simulink library "mssSimulink"  (R2024a)
settings: Solver=ode45  StartTime=0.0  StopTime=10.0  RelTol=1e-3
undefined symbols (not defined in the file): ABC, CN_data, CX_data, CY_data, D, G, Hoerner, K_supply, kt2ms, MA, magnitude, MRB, pathlength, RAO_Amp, RAO_Dir, RAO_Freq, RAO_Phase, RAO_Vel, RAO_yaw_back, RAO_yaw_quant, RAO_yaw_quantization_flag, rho_a, slcm, T_supply, table, vessel, vesselABC
libraries: $bdroot x99, simulink x13
(part 3 of 9)

== system mssSimulink/Hydrodynamics/Motion RAO (U=0) ==
  eta LF : Inport
  Waves : Inport  Port=2
  6DOF rotation matrix in yaw : Subsystem
  Bus Selector : BusSelector  OutputSignals=Psi,Wavenum,Omega,Phase,Zeta_a
  Clock : Clock
  Output smoothing : Subsystem
  "Position phase " : $bdroot/Modelling/Environmental Loads/Utilities/Position phase
  Product1 : Product  Inputs=**  SaturateOnIntegerOverflow=on  OutDataTypeStr=Inherit: Same as first input
  Sum : Sum  Inputs=-++  SaturateOnIntegerOverflow=on
  Wave component loop : Subsystem  TreatAsAtomicUnit=on
  Width : Width  DataType=int32
  "Yaw quantizer " : $bdroot/Modelling/Environmental Loads/Utilities/Yaw quantizer  quant_flag=RAO_yaw_quantization_flag  quant=RAO_yaw_quant  back=RAO_yaw_back
  "[-inf inf] to [-pi pi] " : $bdroot/Utilities/Math Operations/[-inf inf] to [-pi pi]
  yaw angle : Selector  InputPortWidth=6  IndexOptions=Index vector (dialog)  Indices=6  OutputSizes=1
  eta WF : Outport
  nu WF : Outport  Port=2
  nu_dot WF : Outport  Port=3
  wires:
  Output smoothing/1("eta_h WF ") -> 6DOF rotation matrix in yaw/2(V)
  Wave component loop/4(nu_dot rate) -> Output smoothing/4(nu_dot rate)
  Wave component loop/1(eta_h WF) -> Output smoothing/1(eta_h WF)
  Output smoothing/3(nu_dot WF) -> nu_dot WF/1
  Output smoothing/2(nu WF) -> nu WF/1
  eta LF/1 -> yaw angle/1, "Position phase "/3
  Bus Selector/2 -> "Position phase "/2  "<Wavenum>"
  Bus Selector/4 -> Sum/3  "<Phase>"
  Waves/1 -> Bus Selector/1
  Product1/1 -> Sum/2
  Bus Selector/1 -> "Position phase "/1, "Yaw quantizer "/2  "<Psi>"
  Clock/1 -> Product1/2
  yaw angle/1 -> 6DOF rotation matrix in yaw/1(psi), "Yaw quantizer "/1
  Bus Selector/3 -> Width/1, Wave component loop/3(Omega), Product1/1  "<Omega>"
  6DOF rotation matrix in yaw/1(R(psi)*V) -> eta WF/1
  Sum/1 -> Wave component loop/4(Phase_tot)  "Phase_tot"
  Bus Selector/5 -> Wave component loop/5(Zeta_a)  "<Zeta_a>"
  Width/1 -> Wave component loop/1(number of iterations)
  Wave component loop/2(nu WF) -> Output smoothing/2("nu WF ")
  Wave component loop/3(nu_dot WF) -> Output smoothing/3("nu_dot WF ")
  "Yaw quantizer "/1 -> "[-inf inf] to [-pi pi] "/1
  "[-inf inf] to [-pi pi] "/1 -> Wave component loop/2(Psi_r)
  "Position phase "/1 -> Sum/1

== system mssSimulink/Hydrodynamics/WD for heading1 ==
  psi : Inport
  psi_wave : Inport  Port=2
  Omega : Inport  Port=3
  Zeta_a : Inport  Port=4
  U : Inport  Port=5
  Sum1 : Sum  Inputs=-+|
  Wave component loop : Subsystem  TreatAsAtomicUnit=on
  Width : Width  DataType=int32
  tau_WD : Outport
  wires:
  Width/1 -> Wave component loop/1(number of iterations)
  psi_wave/1 -> Sum1/2
  Omega/1 -> Wave component loop/3(Omega), Width/1
  Zeta_a/1 -> Wave component loop/4(Zeta_a)
  Sum1/1 -> Wave component loop/2(Psi_r)
  Wave component loop/1(tau_WD) -> tau_WD/1
  U/1 -> Wave component loop/5(U)
  psi/1 -> Sum1/1  "psi"

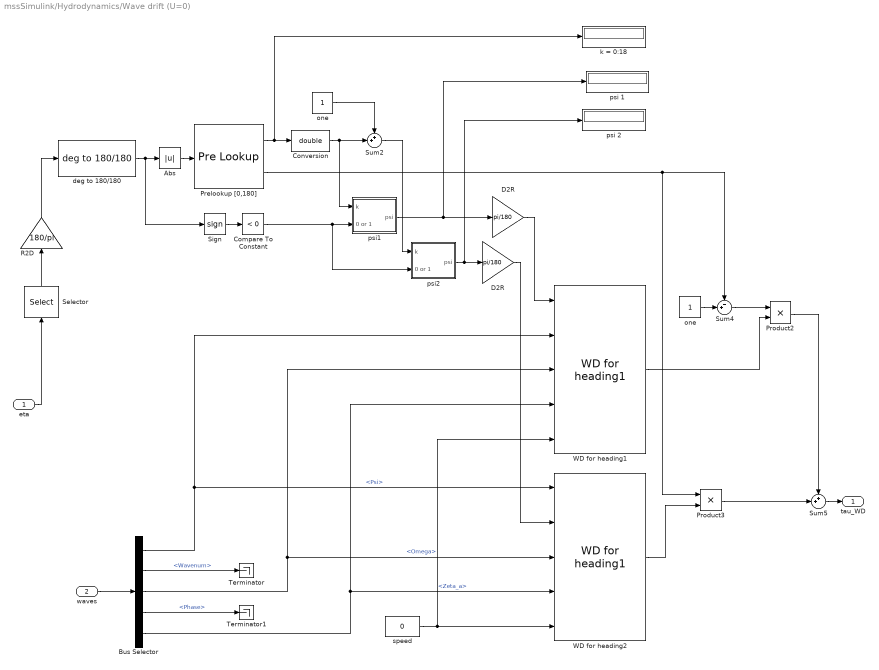
== system mssSimulink/Hydrodynamics/Wave drift (U=0) ==
  eta : Inport
  waves : Inport  Port=2
  Abs : Abs
  Bus Selector : BusSelector  OutputSignals=Psi,Wavenum,Omega,Phase,Zeta_a
  Compare To Constant : simulink/Logic and Bit Operations/Compare To Constant  relop=<  const=0  OutDataTypeStr=uint8  ZeroCross=off
  Conversion : DataTypeConversion  OutDataTypeStr=double  SaturateOnIntegerOverflow=off  RndMeth=Floor
  D2R : Gain  Gain=pi/180
  "D2R " : Gain  Gain=pi/180
  Prelookup [0,180] : PreLookup  BreakpointsData=[0:10:180]  IndexSearchMethod=Evenly spaced points  BeginIndexSearchUsingPreviousIndexResult=on
  Product2 : Product  RndMeth=Zero
  Product3 : Product  RndMeth=Zero
  R2D : Gain  Gain=180/pi
  Selector : Selector  InputPortWidth=6  IndexOptions=Index vector (dialog)  Indices=[6]  OutputSizes=1
  Sign : Signum
  Sum2 : Sum  Inputs=++|
  Sum4 : Sum  Inputs=-+|
  Sum5 : Sum  Inputs=++|
  Terminator : Terminator
  Terminator1 : Terminator
  "WD for heading1 " : $bdroot/Hydrodynamics/WD for heading1  ForceRAO_Freq=vessel.forceRAO.w  WD_Freq=vessel.driftfrc.w  RAO_Vel=vessel.velocities  ForceRAO_Amp=vessel.forceRAO.amp  ForceRAO_Phase=vessel.forceRAO.phase  WD_Amp=vessel.driftfrc.amp  RAO_add_omega_0=on  RAO_add_omega_inf=on
  "WD for heading2 " : $bdroot/Hydrodynamics/WD for heading1  ForceRAO_Freq=vessel.forceRAO.w  WD_Freq=vessel.driftfrc.w  RAO_Vel=vessel.velocities  ForceRAO_Amp=vessel.forceRAO.amp  ForceRAO_Phase=vessel.forceRAO.phase  WD_Amp=vessel.driftfrc.amp  RAO_add_omega_0=on  RAO_add_omega_inf=on
  "deg to 180/180 " : $bdroot/Utilities/Math Operations/deg to 180//180
  k = 0:18 : Display
  one : Constant
  "one " : Constant
  psi 1 : Display
  psi 2 : Display
  psi1 : Subsystem
  psi2 : Subsystem
  speed : Constant  Value=0
  tau_WD : Outport
  wires:
  "WD for heading2 "/1 -> Product3/2
  eta/1 -> Selector/1
  "one "/1 -> Sum4/2
  Sum4/1 -> Product2/1
  "WD for heading1 "/1 -> Product2/2
  Product3/1 -> Sum5/2
  Product2/1 -> Sum5/1
  Prelookup [0,180]/1 -> Conversion/1, k = 0:18/1
  one/1 -> Sum2/1
  Sum2/1 -> psi2/1(k)
  "deg to 180/180 "/1 -> Abs/1, Sign/1
  Abs/1 -> Prelookup [0,180]/1
  Sign/1 -> Compare To Constant/1
  Compare To Constant/1 -> psi1/2(0 or 1), psi2/2(0 or 1)
  psi1/1(psi) -> D2R/1, psi 1/1
  Prelookup [0,180]/2 -> Product3/1, Sum4/1
  Conversion/1 -> Sum2/2, psi1/1(k)
  psi2/1(psi) -> "D2R "/1, psi 2/1
  waves/1 -> Bus Selector/1
  Sum5/1 -> tau_WD/1
  Selector/1 -> R2D/1
  R2D/1 -> "deg to 180/180 "/1
  speed/1 -> "WD for heading2 "/5, "WD for heading1 "/5
  Bus Selector/3 -> "WD for heading2 "/3, "WD for heading1 "/3  "<Omega>"
  Bus Selector/5 -> "WD for heading2 "/4, "WD for heading1 "/4  "<Zeta_a>"
  Bus Selector/2 -> Terminator/1  "<Wavenum>"
  Bus Selector/1 -> "WD for heading1 "/2, "WD for heading2 "/1  "<Psi>"
  Bus Selector/4 -> Terminator1/1  "<Phase>"
  D2R/1 -> "WD for heading1 "/1
  "D2R "/1 -> "WD for heading2 "/2

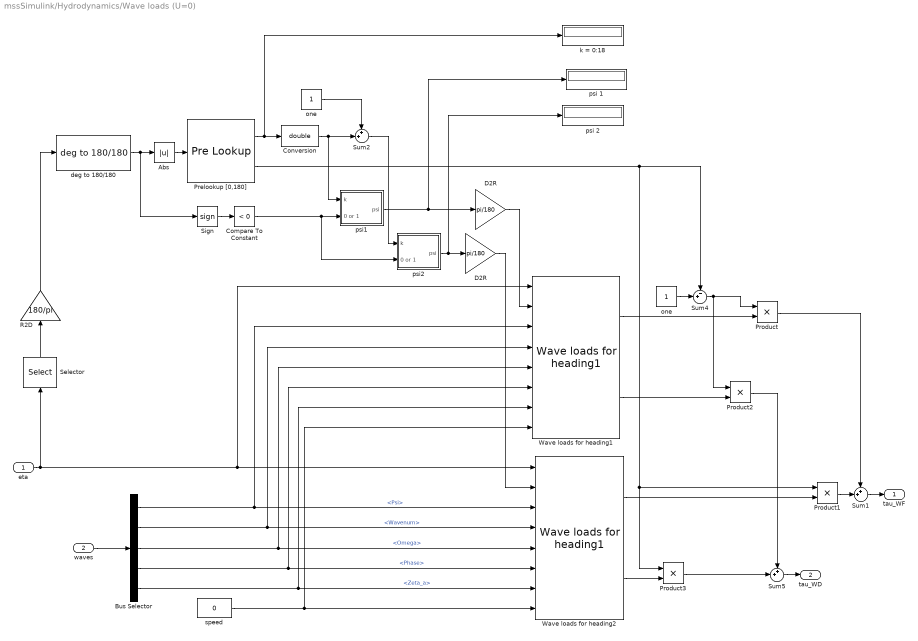
== system mssSimulink/Hydrodynamics/Wave loads (U=0) ==
  eta : Inport
  waves : Inport  Port=2
  Abs : Abs
  Bus Selector : BusSelector  OutputSignals=Psi,Wavenum,Omega,Phase,Zeta_a
  Compare To Constant : simulink/Logic and Bit Operations/Compare To Constant  relop=<  const=0  OutDataTypeStr=uint8  ZeroCross=off
  Conversion : DataTypeConversion  OutDataTypeStr=double  SaturateOnIntegerOverflow=off  RndMeth=Floor
  D2R : Gain  Gain=pi/180
  "D2R " : Gain  Gain=pi/180
  Prelookup [0,180] : PreLookup  BreakpointsData=[0:10:180]  IndexSearchMethod=Evenly spaced points  BeginIndexSearchUsingPreviousIndexResult=on
  Product{,1..3} (4 alike) : Product  RndMeth=Zero
  R2D : Gain  Gain=180/pi
  Selector : Selector  InputPortWidth=6  IndexOptions=Index vector (dialog)  Indices=[6]  OutputSizes=1
  Sign : Signum
  Sum1 : Sum  Inputs=++|
  Sum2 : Sum  Inputs=++|
  Sum4 : Sum  Inputs=-+|
  Sum5 : Sum  Inputs=++|
  "Wave loads for heading1 " : $bdroot/Hydrodynamics/Wave loads for heading1  ForceRAO_Freq=vessel.forceRAO.w  WD_Freq=vessel.driftfrc.w  RAO_Vel=vessel.velocities  ForceRAO_Amp=vessel.forceRAO.amp  ForceRAO_Phase=vessel.forceRAO.phase  WD_Amp=vessel.driftfrc.amp  RAO_add_omega_0=on  RAO_add_omega_inf=on
  Wave loads for heading2 : $bdroot/Hydrodynamics/Wave loads for heading1  ForceRAO_Freq=vessel.forceRAO.w  WD_Freq=vessel.driftfrc.w  RAO_Vel=vessel.velocities  ForceRAO_Amp=vessel.forceRAO.amp  ForceRAO_Phase=vessel.forceRAO.phase  WD_Amp=vessel.driftfrc.amp  RAO_add_omega_0=on  RAO_add_omega_inf=on
  "deg to 180/180 " : $bdroot/Utilities/Math Operations/deg to 180//180
  k = 0:18 : Display
  one : Constant
  "one " : Constant
  psi 1 : Display
  psi 2 : Display
  psi1 : Subsystem
  psi2 : Subsystem
  speed : Constant  Value=0
  tau_WF : Outport
  tau_WD : Outport  Port=2
  wires:
  R2D/1 -> "deg to 180/180 "/1
  Selector/1 -> R2D/1
  Sum5/1 -> tau_WD/1
  waves/1 -> Bus Selector/1
  Sum1/1 -> tau_WF/1
  "D2R "/1 -> Wave loads for heading2/2
  D2R/1 -> "Wave loads for heading1 "/2
  psi2/1(psi) -> psi 2/1, "D2R "/1
  Conversion/1 -> psi1/1(k), Sum2/2
  Prelookup [0,180]/2 -> Sum4/1, Product1/1, Product3/1
  psi1/1(psi) -> psi 1/1, D2R/1
  Compare To Constant/1 -> psi2/2(0 or 1), psi1/2(0 or 1)
  Sign/1 -> Compare To Constant/1
  Abs/1 -> Prelookup [0,180]/1
  "deg to 180/180 "/1 -> Sign/1, Abs/1
  Sum2/1 -> psi2/1(k)
  one/1 -> Sum2/1
  Prelookup [0,180]/1 -> k = 0:18/1, Conversion/1
  Product2/1 -> Sum5/1
  Product3/1 -> Sum5/2
  "Wave loads for heading1 "/2 -> Product2/2
  Sum4/1 -> Product2/1, Product/1
  "one "/1 -> Sum4/2
  Product1/1 -> Sum1/2
  Product/1 -> Sum1/1
  "Wave loads for heading1 "/1 -> Product/2
  Bus Selector/5 -> Wave loads for heading2/7, "Wave loads for heading1 "/7  "<Zeta_a>"
  Bus Selector/4 -> Wave loads for heading2/6, "Wave loads for heading1 "/6  "<Phase>"
  Bus Selector/3 -> Wave loads for heading2/5, "Wave loads for heading1 "/5  "<Omega>"
  Bus Selector/2 -> Wave loads for heading2/4, "Wave loads for heading1 "/4  "<Wavenum>"
  Bus Selector/1 -> Wave loads for heading2/3, "Wave loads for heading1 "/3  "<Psi>"
  eta/1 -> Selector/1, Wave loads for heading2/1, "Wave loads for heading1 "/1
  Wave loads for heading2/2 -> Product3/2
  Wave loads for heading2/1 -> Product1/2
  speed/1 -> Wave loads for heading2/8, "Wave loads for heading1 "/8

== system mssSimulink/Hydrodynamics/Wave loads (U>0) ==
  eta : Inport
  waves : Inport  Port=2
  U : Inport  Port=3
  Abs : Abs
  Conversion : DataTypeConversion  OutDataTypeStr=double  SaturateOnIntegerOverflow=off  RndMeth=Floor
  Prelookup : PreLookup  BreakpointsData=vessel.velocities  IndexSearchMethod=Linear search  BeginIndexSearchUsingPreviousIndexResult=on
  Product{,1..3} (4 alike) : Product  RndMeth=Zero
  Sum1 : Sum  Inputs=++|
  Sum2 : Sum  Inputs=++|
  Sum4 : Sum  Inputs=-+|
  Sum5 : Sum  Inputs=++|
  Wave loads U = U1 : Subsystem
  Wave loads U = U2 : Subsystem
  one : Constant
  "one " : Constant
  tau_WF : Outport
  tau_WD : Outport  Port=2
  wires:
  waves/1 -> Wave loads U = U1/2(waves), Wave loads U = U2/2(waves)
  eta/1 -> Wave loads U = U1/1(eta), Wave loads U = U2/1(eta)
  Conversion/1 -> Sum2/2, Wave loads U = U1/3(U_idx)
  Abs/1 -> Prelookup/1
  one/1 -> Sum2/1
  Prelookup/1 -> Conversion/1
  Sum2/1 -> Wave loads U = U2/3(U_idx)
  Sum5/1 -> tau_WD/1
  Sum1/1 -> tau_WF/1
  Prelookup/2 -> Product1/1, Product3/1, Sum4/1
  Product2/1 -> Sum5/1
  Product3/1 -> Sum5/2
  Sum4/1 -> Product2/1, Product/1
  "one "/1 -> Sum4/2
  Product1/1 -> Sum1/2
  Product/1 -> Sum1/1
  Wave loads U = U1/1(tau_WF) -> Product/2
  Wave loads U = U2/2(tau_WD) -> Product3/2
  Wave loads U = U2/1(tau_WF) -> Product1/2
  Wave loads U = U1/2(tau_WD) -> Product2/2
  U/1 -> Abs/1

== system mssSimulink/Hydrodynamics/Wave loads for heading1 ==
  eta : Inport
  psi : Inport  Port=2
  psi_wave : Inport  Port=3
  wavenum : Inport  Port=4
  Omega : Inport  Port=5
  Phase : Inport  Port=6
  Zeta_a : Inport  Port=7
  U : Inport  Port=8
  Clock : Clock
  "Position phase " : $bdroot/Modelling/Environmental Loads/Utilities/Position phase
  Product1 : Product  Inputs=**  SaturateOnIntegerOverflow=on  OutDataTypeStr=Inherit: Same as first input
  Sum : Sum  Inputs=-++  SaturateOnIntegerOverflow=on
  Sum1 : Sum  Inputs=-+|
  Wave component loop : Subsystem  TreatAsAtomicUnit=on
  Width : Width  DataType=int32
  tau_WF : Outport
  tau_WD : Outport  Port=2
  wires:
  psi/1 -> Sum1/1  "psi"
  U/1 -> Wave component loop/6(U)
  Wave component loop/2(tau_WD) -> tau_WD/1
  Sum1/1 -> Wave component loop/2(Psi_r)
  Zeta_a/1 -> Wave component loop/5(Zeta_a)
  Phase/1 -> Sum/3
  Omega/1 -> Width/1, Wave component loop/3(Omega), Product1/1
  wavenum/1 -> "Position phase "/2
  psi_wave/1 -> Sum1/2, "Position phase "/1
  eta/1 -> "Position phase "/3
  Wave component loop/1(tau_WF) -> tau_WF/1
  Product1/1 -> Sum/2
  Clock/1 -> Product1/2
  Sum/1 -> Wave component loop/4(Phase_tot)  "Phase_tot"
  Width/1 -> Wave component loop/1(number of iterations)
  "Position phase "/1 -> Sum/1

== system mssSimulink/Hydrodynamics/zero-speed viiscous roll damping ==
  p : Inport
  A44 : Constant  Value=vesselABC.A44(:,:,1)
  B44 : Constant  Value=vesselABC.B44(:,:,1)
  B44_inf : Constant  Value=vesselABC.B44_inf(1)
  C44 : Constant  Value=vesselABC.C44(:,:,1)
  D44 : Constant  Value=vesselABC.D44(:,:,1)
  Integrator : Integrator
  Math Function : Math  Operator=transpose  SignedPower=on
  Product{,1..2,4} (4 alike) : Product  Multiplication=Matrix(*)  RndMeth=Zero
  Product3 : Product  RndMeth=Zero
  Sum : Sum  Inputs=++|
  Sum1 : Sum  Inputs=|++
  Sum2 : Sum  Inputs=++|
  K_visc : Outport
  wires:
  Math Function/1 -> Product2/1
  B44/1 -> Product1/1
  Sum1/1 -> Sum2/2
  Product2/1 -> Sum1/1
  Product3/1 -> Sum1/2
  D44/1 -> Product3/1
  C44/1 -> Math Function/1
  Sum/1 -> Integrator/1
  Product/1 -> Sum/2
  Product1/1 -> Sum/1
  A44/1 -> Product/1
  Integrator/1 -> Product2/2, Product/2
  p/1 -> Product3/2, Product1/2, Product4/2
  Sum2/1 -> K_visc/1
  B44_inf/1 -> Product4/1
  Product4/1 -> Sum2/1

== system mssSimulink/Marine craft models/4-DOF naval vessel ==
  tau (X,Y,K,N) : Inport
  Initial conditions (u,v,p,r,phi,psi) : Constant  Value=x0
  Integrator : Integrator  InitialConditionSource=external  InitialCondition=[1 1]  UpperSaturationLimit=10  LowerSaturationLimit=-10
  Mux1 : Mux  Inputs=2
  Selector : Selector  InputPortWidth=6  IndexOptions=Index vector (dialog)  Indices=[1 2 3 4]  OutputSizes=1
  Selector1 : Selector  InputPortWidth=6  IndexOptions=Index vector (dialog)  Indices=[5 6]  OutputSizes=1
  navalvessel.m : MATLABFcn  MATLABFcn=feval('navalvessel',u(1:6),u(7:10))  OutputDimensions=6  Output1D=off
  eta (phi,psi) : Outport  VectorParamsAs1DForOutWhenUnconnected=off
  nu (u,v,p,r) : Outport  Port=2  VectorParamsAs1DForOutWhenUnconnected=off
  wires:
  Selector/1 -> nu (u,v,p,r)/1
  Selector1/1 -> eta (phi,psi)/1
  Integrator/1 -> Selector1/1, Selector/1, Mux1/1
  Initial conditions (u,v,p,r,phi,psi)/1 -> Integrator/2
  tau (X,Y,K,N)/1 -> Mux1/2
  navalvessel.m/1 -> Integrator/1
  Mux1/1 -> navalvessel.m/1

== system mssSimulink/Marine craft models/6-DOF semisub ==
  tau : Inport
  nu_c : Inport  Port=2
  "6 DOF Eqs. of motion " : $bdroot/Modelling/Kinetics /6 DOF Eqs. of motion  CoriolisOnOff=on  nu0=[0 0 0 0 0 0]  eta0=[0 0 0 0 0 0]
      link override 6 DOF Coriolis forces: SourceBlock=mssSimulink/Modelling/Kinetics /Support/6 DOF Coriolis forces
      link override 6 DOF Coriolis forces1: SourceBlock=mssSimulink/Modelling/Kinetics /Support/6 DOF Coriolis forces
      link override Euler angles to rotation matrix: SourceBlock=mssSimulink/Modelling/Kinematics/Euler angles to rotation matrix
  Constant : Constant  Value=MRB
  "Constant " : Constant  Value=MA
  D : Gain  Gain=D  Multiplication=Matrix(K*u)  SaturateOnIntegerOverflow=on  OutDataTypeStr=Inherit: Same as input  ParamDataTypeStr=Inherit: Same as input
  G : Gain  Gain=G  Multiplication=Matrix(K*u)  SaturateOnIntegerOverflow=on  OutDataTypeStr=Inherit: Same as input  ParamDataTypeStr=Inherit: Same as input
  Sum : Sum  Inputs=+--  InputSameDT=on  SaturateOnIntegerOverflow=on  OutDataTypeStr=Inherit: Same as first input
  Sum1 : Sum  Inputs=-+|  SaturateOnIntegerOverflow=on
  eta : Outport  InitialOutput=0  VectorParamsAs1DForOutWhenUnconnected=off
  nu : Outport  Port=2  InitialOutput=0  VectorParamsAs1DForOutWhenUnconnected=off
  wires:
  "Constant "/1 -> "6 DOF Eqs. of motion "/2
  Sum/1 -> "6 DOF Eqs. of motion "/3
  Sum1/1 -> D/1
  nu_c/1 -> Sum1/1, "6 DOF Eqs. of motion "/4
  Constant/1 -> "6 DOF Eqs. of motion "/1
  "6 DOF Eqs. of motion "/1 -> eta/1, G/1
  "6 DOF Eqs. of motion "/2 -> Sum1/2, nu/1
  G/1 -> Sum/2
  D/1 -> Sum/3
  tau/1 -> Sum/1

== system mssSimulink/Marine craft models/6-DOF supply vessel interface ==
  tau : Inport
  3 to 6 DOF : $bdroot/Modelling/Kinetics /Support/3 to 6 DOF  SystemSampleTime=-1  VariantActivationTime=update diagram  AllowFlexibleInterface=on  Latency=0  AutoFrameSizeCalculation=off
  3 to 6 DOF1 : $bdroot/Modelling/Kinetics /Support/3 to 6 DOF  SystemSampleTime=-1  VariantActivationTime=update diagram  AllowFlexibleInterface=on  Latency=0  AutoFrameSizeCalculation=off
  6 to 3 DOF1 : Selector  InputPortWidth=6  IndexOptions=Index vector (dialog)  Indices=[1 2 6]  OutputSizes=1
  Supply vessel : $bdroot/Marine craft models/Supply vessel  D=[5.0242e4 0 0; 0 2.7229e5 -4.3933e6; 0 -4.3933e6 4.1894e8]  Minv=inv( [5.3122e6 0 0; 0 8.2831e6 0; 0 0 3.7454e9] )
  eta : Outport  VectorParamsAs1DForOutWhenUnconnected=off
  nu : Outport  Port=2  VectorParamsAs1DForOutWhenUnconnected=off
  wires:
  3 to 6 DOF1/1 -> nu/1
  tau/1 -> 6 to 3 DOF1/1
  3 to 6 DOF/1 -> eta/1
  6 to 3 DOF1/1 -> Supply vessel/1
  Supply vessel/2 -> 3 to 6 DOF1/1
  Supply vessel/1 -> 3 to 6 DOF/1

== system mssSimulink/Marine craft models/Container ship: L = 175 m ==
  u : Inport
  xo : Inport  Port=2
  Integrator : Integrator  InitialConditionSource=external  InitialCondition=[1 1]  UpperSaturationLimit=10  LowerSaturationLimit=-10
  Mux1 : Mux  Inputs=2
  m-file : MATLABFcn  MATLABFcn=feval(vessmodel,u(1:dimx_model),u(dimx_model+1:length(u)))  Output1D=off
  x : Outport  VectorParamsAs1DForOutWhenUnconnected=off
  wires:
  xo/1 -> Integrator/2
  u/1 -> Mux1/2
  Mux1/1 -> m-file/1
  Integrator/1 -> x/1, Mux1/1
  m-file/1 -> Integrator/1

== system mssSimulink/Marine craft models/CyberShipII ==
  note: etadot
  note: nu_dot
  note: nu
  tau : Inport
  D : Gain  Gain=D  Multiplication=Matrix(K*u)  SaturateOnIntegerOverflow=on  OutDataTypeStr=Inherit: Same as input  ParamDataTypeStr=Inherit: Same as input
  Integrator1 : Integrator
  Integrator2 : Integrator
  Rotation matrix in yaw 1 : $bdroot/Modelling/Kinematics/Rotation matrix in yaw 
  Sum3 : Sum  Inputs=+-  InputSameDT=on  SaturateOnIntegerOverflow=on  OutDataTypeStr=Inherit: Same as first input
  inv(M) : Gain  Gain=inv(M)  Multiplication=Matrix(K*u)  SaturateOnIntegerOverflow=on  OutDataTypeStr=Inherit: Same as input  ParamDataTypeStr=Inherit: Same as input
  psi : Selector  InputPortWidth=3  IndexOptions=Index vector (dialog)  Indices=[3]  OutputSizes=1
  saturation : Subsystem
  eta : Outport  VectorParamsAs1DForOutWhenUnconnected=off
  nu : Outport  Port=2  VectorParamsAs1DForOutWhenUnconnected=off
  wires:
  saturation/1(sat_tau) -> Sum3/1
  psi/1 -> Rotation matrix in yaw 1/1
  Integrator1/1 -> psi/1, eta/1
  Rotation matrix in yaw 1/1 -> Integrator1/1
  inv(M)/1 -> Integrator2/1
  Sum3/1 -> inv(M)/1
  D/1 -> Sum3/2
  Integrator2/1 -> D/1, nu/1, Rotation matrix in yaw 1/2
  tau/1 -> saturation/1(tau)

== system mssSimulink/Marine craft models/Deep submergence rescue vehicle (DSRV.m) ==
  u : Inport
  x0 : Inport  Port=2
  Integrator : Integrator  InitialConditionSource=external  InitialCondition=[1 1]  UpperSaturationLimit=10  LowerSaturationLimit=-10
  MATLAB Function : MATLAB Function  TreatAsAtomicUnit=on
  x : Outport
  U : Outport  Port=2
  wires:
  MATLAB Function/2(U) -> U/1
  x0/1 -> Integrator/2
  MATLAB Function/1(xdot) -> Integrator/1
  Integrator/1 -> x/1, MATLAB Function/1(x)
  u/1 -> MATLAB Function/2(u)

== system mssSimulink/Marine craft models/Large tanker: L = 304 m ==
  u : Inport
  xo : Inport  Port=2
  Integrator : Integrator  InitialConditionSource=external  InitialCondition=[1 1]  UpperSaturationLimit=10  LowerSaturationLimit=-10
  Mux1 : Mux  Inputs=2
  m-file : MATLABFcn  MATLABFcn=feval(vessmodel,u(1:dimx_model),u(dimx_model+1:length(u)))  Output1D=off
  x : Outport  VectorParamsAs1DForOutWhenUnconnected=off
  wires:
  xo/1 -> Integrator/2
  u/1 -> Mux1/2
  Mux1/1 -> m-file/1
  Integrator/1 -> x/1, Mux1/1
  m-file/1 -> Integrator/1

== system mssSimulink/Marine craft models/Mariner class cargo ship (2nd -order) ==
  rudder command : Inport
  Integrator : Integrator
  Ship model : Subsystem
  Sum : Sum  Inputs=|+-  InputSameDT=on  SaturateOnIntegerOverflow=on  OutDataTypeStr=Inherit: Same as first input
  rudder angle saturation : Saturate  UpperLimit=delta_max  LowerLimit=-delta_max
  rudder rate saturation : Saturate  UpperLimit=rate_max  LowerLimit=-rate_max
  heading angle : Outport  VectorParamsAs1DForOutWhenUnconnected=off
  heading rate : Outport  Port=2  VectorParamsAs1DForOutWhenUnconnected=off
  rudder angle : Outport  Port=3  VectorParamsAs1DForOutWhenUnconnected=off
  wires:
  rudder command/1 -> rudder angle saturation/1
  Ship model/1(heading angle) -> heading angle/1
  Ship model/2(heading rate) -> heading rate/1
  Integrator/1 -> Sum/2, Ship model/1(rudder angle), rudder angle/1
  rudder angle saturation/1 -> Sum/1
  Sum/1 -> rudder rate saturation/1
  rudder rate saturation/1 -> Integrator/1

== system mssSimulink/Marine craft models/Mariner class cargo ship (mariner.m) ==
  u : Inport
  x0 : Inport  Port=2
  U0 : Inport  Port=3
  Integrator : Integrator  InitialConditionSource=external  InitialCondition=[1 1]  UpperSaturationLimit=10  LowerSaturationLimit=-10
  MATLAB Function : MATLAB Function  TreatAsAtomicUnit=on
  x : Outport
  U : Outport  Port=2
  wires:
  u/1 -> MATLAB Function/2(u)
  Integrator/1 -> MATLAB Function/1(x), x/1
  MATLAB Function/1(xdot) -> Integrator/1
  x0/1 -> Integrator/2
  MATLAB Function/2(U) -> U/1
  U0/1 -> MATLAB Function/3(U0)

== system mssSimulink/Marine craft models/Naval Postgraduate School AUV (npsAUV.m) ==
  u : Inport
  x0 : Inport  Port=2
  Integrator : Integrator  InitialConditionSource=external  InitialCondition=[1 1]  UpperSaturationLimit=10  LowerSaturationLimit=-10
  MATLAB Function : MATLAB Function  TreatAsAtomicUnit=on
  x : Outport
  U : Outport  Port=2
  wires:
  MATLAB Function/2(U) -> U/1
  x0/1 -> Integrator/2
  MATLAB Function/1(xdot) -> Integrator/1
  Integrator/1 -> x/1, MATLAB Function/1(x)
  u/1 -> MATLAB Function/2(u)

== system mssSimulink/Marine craft models/Otter USV (otter.m) ==
  n : Inport
  mp : Inport  Port=2
  rp : Inport  Port=3
  V_c : Inport  Port=4
  beta_c : Inport  Port=5
  x0 : Inport  Port=6
  Demux : Demux  Outputs=2
  Integrator : Integrator  InitialConditionSource=external  InitialCondition=[1 1]  UpperSaturationLimit=10  LowerSaturationLimit=-10
  Mux : Mux  Inputs=2
  Otter USV : MATLAB Function  TreatAsAtomicUnit=on
  Transfer Fcn : TransferFcn  Denominator=[0.1 1]
  Transfer Fcn1 : TransferFcn  Denominator=[0.1 1]
  x : Outport
  U : Outport  Port=2
  wires:
  x0/1 -> Integrator/2
  n/1 -> Demux/1
  rp/1 -> Otter USV/4(rp)
  beta_c/1 -> Otter USV/6(beta_c)
  Integrator/1 -> x/1, Otter USV/1(x)
  Otter USV/1(xdot) -> Integrator/1
  mp/1 -> Otter USV/3(mp)
  Otter USV/2(U) -> U/1
  V_c/1 -> Otter USV/5(V_c)
  Demux/1 -> Transfer Fcn1/1
  Demux/2 -> Transfer Fcn/1
  Transfer Fcn/1 -> Mux/2
  Mux/1 -> Otter USV/2(n)
  Transfer Fcn1/1 -> Mux/1

== system mssSimulink/Marine craft models/Remus 100 AUV (remus100.m) ==
  u : Inport
  x0 : Inport  Port=2
  Vc : Inport  Port=3
  betaVc : Inport  Port=4
  Integrator : Integrator  InitialConditionSource=external  InitialCondition=[1 1]  UpperSaturationLimit=10  LowerSaturationLimit=-10
  MATLAB Function : MATLAB Function  TreatAsAtomicUnit=on
  x : Outport
  U : Outport  Port=2
  wires:
  MATLAB Function/2(U) -> U/1
  x0/1 -> Integrator/2
  MATLAB Function/1(xdot) -> Integrator/1
  Integrator/1 -> x/1, MATLAB Function/1(x)
  u/1 -> MATLAB Function/2(ui)
  betaVc/1 -> MATLAB Function/4(betaVc)
  Vc/1 -> MATLAB Function/3(Vc)

== system mssSimulink/Marine craft models/Supply vessel ==
  tau : Inport
  D : Gain  Gain=D  Multiplication=Matrix(K*u)  SaturateOnIntegerOverflow=on  OutDataTypeStr=Inherit: Same as input  ParamDataTypeStr=Inherit: Same as input
  Integrator : Integrator
  Integrator1 : Integrator
  Minv : Gain  Gain=Minv  Multiplication=Matrix(K*u)  SaturateOnIntegerOverflow=on  OutDataTypeStr=Inherit: Same as input  ParamDataTypeStr=Inherit: Same as input
  "Rotation matrix in yaw " : $bdroot/Modelling/Kinematics/Rotation matrix in yaw 
  Sum : Sum  Inputs=+-  InputSameDT=on  SaturateOnIntegerOverflow=on  OutDataTypeStr=Inherit: Same as first input
  yaw angle : Fcn  Expr=u(3)
  eta : Outport  InitialOutput=0  VectorParamsAs1DForOutWhenUnconnected=off
  nu : Outport  Port=2  InitialOutput=0  VectorParamsAs1DForOutWhenUnconnected=off
  wires:
  Integrator1/1 -> eta/1, yaw angle/1  "eta"
  Integrator/1 -> nu/1, "Rotation matrix in yaw "/2, D/1  "nu"
  yaw angle/1 -> "Rotation matrix in yaw "/1  "psi"
  "Rotation matrix in yaw "/1 -> Integrator1/1
  tau/1 -> Sum/1
  Minv/1 -> Integrator/1
  Sum/1 -> Minv/1
  D/1 -> Sum/2

== system mssSimulink/Marine craft models/Tanker (1st-order) ==
  rudder command : Inport
  Integrator : Integrator
  Ship model : Subsystem
  Sum : Sum  Inputs=|+-  InputSameDT=on  SaturateOnIntegerOverflow=on  OutDataTypeStr=Inherit: Same as first input
  rudder angle saturation : Saturate  UpperLimit=delta_max  LowerLimit=-delta_max
  rudder rate saturation : Saturate  UpperLimit=rate_max  LowerLimit=-rate_max
  heading angle : Outport  VectorParamsAs1DForOutWhenUnconnected=off
  heading rate : Outport  Port=2  VectorParamsAs1DForOutWhenUnconnected=off
  rudder angle : Outport  Port=3  VectorParamsAs1DForOutWhenUnconnected=off
  wires:
  Ship model/2(heading rate) -> heading rate/1
  Ship model/1(heading angle) -> heading angle/1
  Integrator/1 -> Sum/2, Ship model/1(rudder angle), rudder angle/1
  rudder angle saturation/1 -> Sum/1
  Sum/1 -> rudder rate saturation/1
  rudder rate saturation/1 -> Integrator/1
  rudder command/1 -> rudder angle saturation/1

== system mssSimulink/Marine craft models/Tanker (2nd-order) ==
  rudder command : Inport
  Integrator : Integrator
  Ship model : Subsystem
  Sum : Sum  Inputs=|+-  InputSameDT=on  SaturateOnIntegerOverflow=on  OutDataTypeStr=Inherit: Same as first input
  rudder angle saturation : Saturate  UpperLimit=delta_max  LowerLimit=-delta_max
  rudder rate saturation : Saturate  UpperLimit=rate_max  LowerLimit=-rate_max
  heading angle : Outport  VectorParamsAs1DForOutWhenUnconnected=off
  heading rate : Outport  Port=2  VectorParamsAs1DForOutWhenUnconnected=off
  rudder angle : Outport  Port=3  VectorParamsAs1DForOutWhenUnconnected=off
  wires:
  Ship model/1(heading angle) -> heading angle/1
  Ship model/2(heading rate) -> heading rate/1
  Integrator/1 -> Sum/2, Ship model/1(rudder angle), rudder angle/1
  rudder angle saturation/1 -> Sum/1
  Sum/1 -> rudder rate saturation/1
  rudder rate saturation/1 -> Integrator/1
  rudder command/1 -> rudder angle saturation/1

== system mssSimulink/Modelling/Control Surfaces ==
  Fin/Rudder Machinery : Subsystem  mask(Rudder Machinery){Dmax=[], Dvmax=[], tc=[]}
      mask prompts: Dmax "Max. Rudder Angle (rad):"; Dvmax "Max. Rudder Rate (rad/sec.):"; tc "Time constant (sec):"
      mask help:
      | Model of van Amerongen for rudder machiery
      | Copyright (C) 2005 NTNU
      | Author: Tristan Perez
      mask Help: Rudder machinery model of Van Amerongen accounting for saturation and rate limit.
  Rudder : Subsystem  mask(Rudder Model){LCG=[], VCG=[], sp=[], ar=[], A=[], dCL=[], CD0=[], stall=[], rho=1025}
      mask prompts: LCG "LCG  [m]:"; VCG "VCG [m]:"; sp "Span [m]:"; ar "Aspect ratio:"; A "Area (m^2):"; dCL "dCL/dalpha _e   [1/rad] (deriv of non dimm lift CL(alpha_e)):"; CD0 "CD0 (non-dim Drag @ zero angle of attack):"; stall "Stall angle [rad]:"; rho "Water density  [Kg/m^3]:"
      mask help:
      | Model to generate forces and moments due to rudder action as a control surface.
      | Copyright (C) 2005 NTNU
      | Author: Tristan Perez
      mask Help:
      | This block gives the forces (N) and moments (Nm) in 4-DOF
      |  generated by the rudder.   The inputs of the block are the  effective  angle of attack  "alpha_eff"and  the average speed of the fluid over the rudder "V".
      | "LCG " is the longitudinal
      |  position of the centre of gravity
      | (distance from along the center line from the rudder stock to the CG.) "VCG" is the
      | vertical center of gravity (distance from the base line to GC.)
      | The lift generated is linear until  the stall angle is reached, where the lift saturates.
      | 
      | The units of the angles is in rad and the dCL/dalpha _e   shoudl have units of 1/rad.
  Rudder forces 4-DOF : Subsystem  mask(Rudder forces){rr=[], LCG=[]}
      mask prompts: rr "Rr  (distance CG to CP) [m]:"; LCG "LCG [m]:"
      mask help:
      | This block calculates the forces and moments on the hull in 4-DOF
      | generated by a rudder.
      | Copyright (C) 2005 NTNU
      | Author: Tristan Perez
      mask Help:
      | Lift and  drag are the hydrodynamic forces generated by the rudder hydrofoil.
      | Positive eff. angle of attack produces negative roll motion (roll to port) and
      | negative yaw angle (turn to port).
      |  Rr is the distance from the center of pressure (CP)
      | of the rudder to the CG.  LCG is the lateral CG, i.e the distance from the rudder
      | stock to CG (the AP (aft perpendicular) is assumed on the rudder stock rather
      |  than on the intersection of waterline and the transom.)
  Stabilizer Fins forces 4-DOF : Subsystem  mask(Stabilizer Fins){B=[], rf=[], FCG=[]}
      mask prompts: B "Tilt angle (rad):"; rf "Rf [m]:"; FCG "Dist Fwrd CG (FCG) [m]:"
      mask help:
      | This block calculates the forces and moments on the hull in 4-DOF
      | generated by a pair of fin stabilizers.
      | Copyright (C) 2005 NTNU
      |  Author: Tristan Perez
      mask init:
      | sinB = sin(B);
      mask Help:
      | Nf and Tf are the hydrodynamic forces normal and tangential to the fin.
      | The tilt angle of a  fin  is considered zero if the fins are
      | parallel to the waterline and pi/2 if they are in a rudder-like position.
      | RF is the effective radius to calculate the moments produced by of the fins
      | with respect to the CG.
      | 
      | Positive fin mechanical angle produces negative roll motion (roll to port).
      | The fin mechanical angle is positive  when starborad fin leading edge moves
      | up and trailing edge moves down, while the port fin moves in the opposite way.
      |  If the fins are forward from CG then FCG > 0, and  positive fin
      | mechanical angles induce a positve yaw moment (turn towards starboard).
      | If FCG < 0   positive fin mechanical angles
      | induce a negative  yaw moment (turn towards port.)
  Steady State Hydrofoil : Subsystem  mask(Hydrofoil){ar=[], A=[], CLAE=, AE=[], CD0=[], rho=[]}
      mask prompts: ar "Aspect ratio:"; A "Area (m^2):"; CLAE "CL(Ang)  Vector:"; AE "Ang   Vector (rad):"; CD0 "CD0 (non-dim Drag @ zero angle of attack):"; rho "Water density  [Kg/m^3]:"
      mask help:
      | Model of a hydrofoil.
      |
      | Inputs:
      | Ang --Effective Angle of Attack    (rad)
      | Vf -- Fluid velocity (m7sec)
      |
      | Outputs:
      | L --Lift force normal to the fluid velocity (N)
      | D -- Drag force in the direction of the fluid (N)
      | N --force normal to the foil (N)
      | T--Force tangential to the foil (N)
      |
      | Parameters: See help.
      | Dpendencies MSS/Toolboxes: None
      | Model Limitations: See Help.
      |
      | Copyright (C) 2005  NTNU
      | Author: Tristan Perez
      mask init:
      | AM = max(AE);
      mask Help: web(['file:///' which('Help_Steady_State_Hydrofoil.htm')], '-helpbrowser');
